simulink model "CompoundGeneratorModel"  (R2023b)
settings: Solver=VariableStepAuto  StartTime=0.0  StopTime=10.0  RelTol=1e-3
libraries: spsDCMachineLib x1, spsDCVoltageSourceLib x1, spsSeriesRLCBranchLib x1, sps_lib x1
settings Model: Creator=bolt  LastModifiedBy=Yunus Emre Turunç
settings SolverCC: AlgebraicLoopSolver=TrustRegion
settings DebuggingCC: UnconnectedInputMsg=warning  UnconnectedOutputMsg=warning  UnconnectedLineMsg=warning
settings ModelReferenceCC: EnableRefExpFcnMdlSchedulingChecks=on

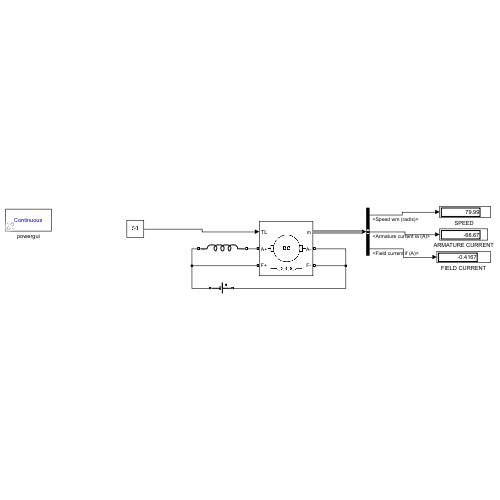
[thumbnail: Simulink's stored preview of the top-level diagram]
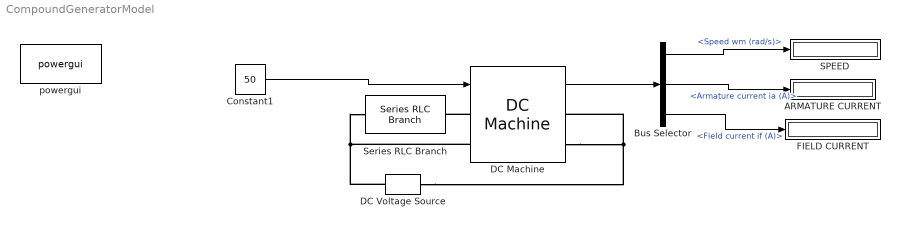
== system CompoundGeneratorModel ==
  ARMATURE CURRENT : Display
  Bus Selector : BusSelector  OutputSignals=Speed wm (rad/s),Armature current ia (A),Field current if (A)
  Constant1 : Constant  Value=50
  DC Machine : spsDCMachineLib/DC Machine  PresetModel=No  MechanicalLoad=Torque TL  FieldType=Wound  ShowDetailedParameters=on  MeasurementBus=off  RLa="[ 0.6  0.012]"  RLf="[ 240  120]"  Laf=1.8  MachineConstant=Torque constant (N.m/A)  Ke=1.8  Kt=1.8  J=1  Bm=0  Tf=0  w0=1  Ifinit=-0.416666666666667  TsPowergui=0  TsBlock=-1
  DC Voltage Source : spsDCVoltageSourceLib/DC Voltage Source  Amplitude=100  Measurements=None
  FIELD CURRENT : Display
  "SPEED " : Display
  Series RLC Branch : spsSeriesRLCBranchLib/Series RLC Branch  LConnTagsString=__new0  RConnTagsString=__new0  BranchType=L  Resistance=1  Inductance=1e-3  SetiL0=off  InitialCurrent=0  Capacitance=1e-6  Setx0=off  InitialVoltage=0  Measurements=None
  powergui : sps_lib/powergui  Priority=1  SimulationMode=Continuous  SampleTime=50e-6  frequency=60  Iterations=50  frequencyindice=0  Pbase=100e6  ErrMax=1e-4  UnitsV=kV  UnitsW=MW  buscounter=0  FunctionMessages=off  echomessages=off  EnableUseOfTLC=off  CurrentSourceSwitches=off  DisableSnubberDevices=off  DisableRonSwitches=off  DisableVfSwitches=off  DisplayEquations=off  AutomaticDiscreteSolvers=off  SolverType=Tustin/Backward Euler (TBE)  Interpol=off  ExternalGateDelay=off  methode=off  Ts=100  x0status=blocks  SPID=on  SwTol=0  HookPort=off  NonlinearTolerance=1e-4  nMaxIteration=100  ContinueOnMaxIteration=off  RestoreLinks=warning  ResistiveCurrentMeasurement=off  Frange=[0:2:500]  Ylog=off  Xlog=on  ShowGrid=off  save=off  variable=ZData  structure=0  ZoomFFT=off  StartTime=0.0  cycles=1  DisplayStyle=1  fundamental=60  FreqAxis=off  MaxFrequency=1000  frequencyindicesteady=1  RmsSteady=1  display=off
  wires:
  Constant1/1 -> DC Machine/1
  DC Machine/1 -> Bus Selector/1
  Bus Selector/1 -> "SPEED "/1  "<Speed wm (rad/s)>"
  Bus Selector/2 -> ARMATURE CURRENT/1  "<Armature current ia (A)>"
  Bus Selector/3 -> FIELD CURRENT/1  "<Field current if (A)>"
  connections:
  DC Machine/LConn1 -- Series RLC Branch/RConn1
  DC Machine/RConn2 -- DC Voltage Source/RConn1 -- DC Machine/RConn1
  DC Voltage Source/LConn1 -- Series RLC Branch/LConn1 -- DC Machine/LConn2
